simulink model "boost_converter_comparison"  (R2026a)
settings: Solver=ode4  StopTime=0.5  FixedStep=1e-05
values from neighbouring files (symbols this model uses):
  Vref = p.Vref    [disturbance_test_script.m]    (also in run_all_controllers.m)
undefined symbols (not defined in the file or in its folder): C, L, rL, Rload, Vin
libraries: fuzblock x2
settings Model: Creator=akash  LastModifiedBy=akash

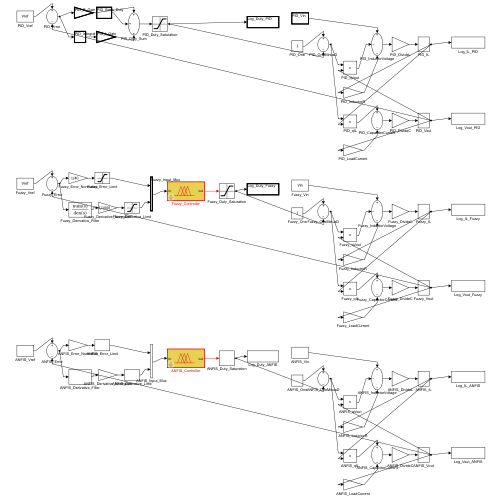
[thumbnail: Simulink's stored preview of the top-level diagram]
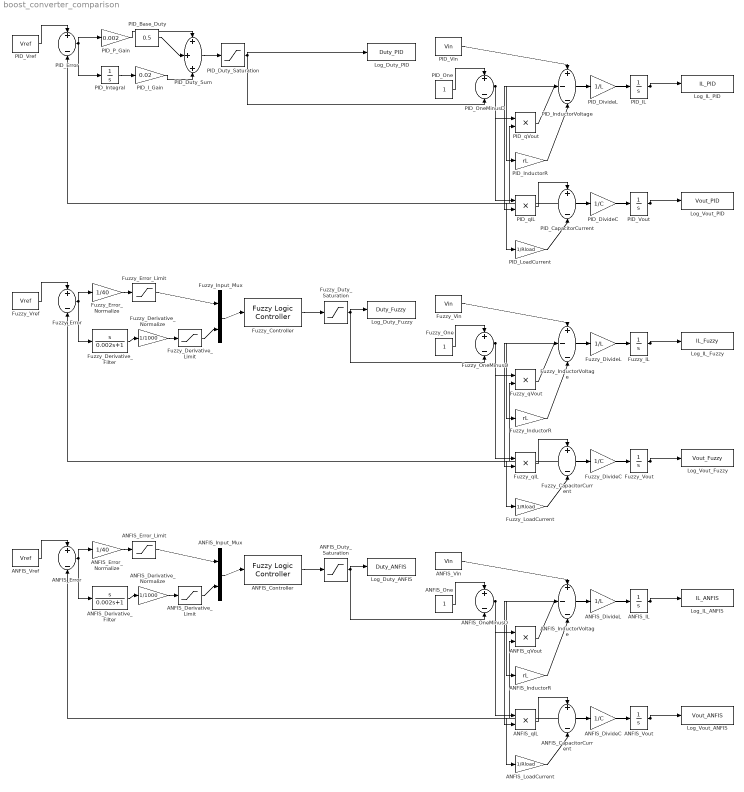
== system boost_converter_comparison ==
  ANFIS_CapacitorCurrent : Sum  Inputs=+-
  ANFIS_Controller : fuzblock/Fuzzy Logic  Controller  FIS=anfisFIS  OutputSampleNumber=101  DataType=double  UseLookupTable=off  NumBreakpoints=10  FuzzifiedInputs=off  RuleFiringStrengths=off  RuleOutputs=off  AggregatedOutputs=off  SimulateUsing=Interpreted execution  OutOfRangeInputValueMessage=warning  NoRuleFiredMessage=warning  EmptyOutputFuzzySetMessage=warning
      settings: LibrarySourceBlock=|
      | fuzblock/Fuzzy Logic
      | Controller
      | with Ruleviewer/Fuzzy Logic
      | Controller
  ANFIS_Derivative_Filter : TransferFcn  Numerator=[1 0]  Denominator=[0.002 1]
  ANFIS_Derivative_Limit : Saturate  UpperLimit=1  LowerLimit=-1
  ANFIS_Derivative_Normalize : Gain  Gain=1/1000
  ANFIS_DivideC : Gain  Gain=1/C
  ANFIS_DivideL : Gain  Gain=1/L
  ANFIS_Duty_Saturation : Saturate  UpperLimit=0.65  LowerLimit=0.35
  ANFIS_Error : Sum  Inputs=+-
  ANFIS_Error_Limit : Saturate  UpperLimit=1  LowerLimit=-1
  ANFIS_Error_Normalize : Gain  Gain=1/40
  ANFIS_IL : Integrator
  ANFIS_InductorR : Gain  Gain=rL
  ANFIS_InductorVoltage : Sum  Inputs=+--
  ANFIS_Input_Mux : Mux  Inputs=2
  ANFIS_LoadCurrent : Gain  Gain=1/Rload
  ANFIS_One : Constant
  ANFIS_OneMinusD : Sum  Inputs=+-
  ANFIS_Vin : Constant  Value=Vin
  ANFIS_Vout : Integrator
  ANFIS_Vref : Constant  Value=Vref
  ANFIS_qIL : Product  Inputs=**
  ANFIS_qVout : Product  Inputs=**
  Fuzzy_CapacitorCurrent : Sum  Inputs=+-
  Fuzzy_Controller : fuzblock/Fuzzy Logic  Controller  FIS=fuzzyFIS  OutputSampleNumber=101  DataType=double  UseLookupTable=off  NumBreakpoints=10  FuzzifiedInputs=off  RuleFiringStrengths=off  RuleOutputs=off  AggregatedOutputs=off  SimulateUsing=Interpreted execution  OutOfRangeInputValueMessage=warning  NoRuleFiredMessage=warning  EmptyOutputFuzzySetMessage=warning
      settings: LibrarySourceBlock=|
      | fuzblock/Fuzzy Logic
      | Controller
      | with Ruleviewer/Fuzzy Logic
      | Controller
  Fuzzy_Derivative_Filter : TransferFcn  Numerator=[1 0]  Denominator=[0.002 1]
  Fuzzy_Derivative_Limit : Saturate  UpperLimit=1  LowerLimit=-1
  Fuzzy_Derivative_Normalize : Gain  Gain=1/1000
  Fuzzy_DivideC : Gain  Gain=1/C
  Fuzzy_DivideL : Gain  Gain=1/L
  Fuzzy_Duty_Saturation : Saturate  UpperLimit=0.65  LowerLimit=0.35
  Fuzzy_Error : Sum  Inputs=+-
  Fuzzy_Error_Limit : Saturate  UpperLimit=1  LowerLimit=-1
  Fuzzy_Error_Normalize : Gain  Gain=1/40
  Fuzzy_IL : Integrator
  Fuzzy_InductorR : Gain  Gain=rL
  Fuzzy_InductorVoltage : Sum  Inputs=+--
  Fuzzy_Input_Mux : Mux  Inputs=2
  Fuzzy_LoadCurrent : Gain  Gain=1/Rload
  Fuzzy_One : Constant
  Fuzzy_OneMinusD : Sum  Inputs=+-
  Fuzzy_Vin : Constant  Value=Vin
  Fuzzy_Vout : Integrator
  Fuzzy_Vref : Constant  Value=Vref
  Fuzzy_qIL : Product  Inputs=**
  Fuzzy_qVout : Product  Inputs=**
  Log_Duty_ANFIS : ToWorkspace  VariableName=Duty_ANFIS  SaveFormat=Timeseries  SampleTime=-1
  Log_Duty_Fuzzy : ToWorkspace  VariableName=Duty_Fuzzy  SaveFormat=Timeseries  SampleTime=-1
  Log_Duty_PID : ToWorkspace  VariableName=Duty_PID  SaveFormat=Timeseries  SampleTime=-1
  Log_IL_ANFIS : ToWorkspace  VariableName=IL_ANFIS  SaveFormat=Timeseries  SampleTime=-1
  Log_IL_Fuzzy : ToWorkspace  VariableName=IL_Fuzzy  SaveFormat=Timeseries  SampleTime=-1
  Log_IL_PID : ToWorkspace  VariableName=IL_PID  SaveFormat=Timeseries  SampleTime=-1
  Log_Vout_ANFIS : ToWorkspace  VariableName=Vout_ANFIS  SaveFormat=Timeseries  SampleTime=-1
  Log_Vout_Fuzzy : ToWorkspace  VariableName=Vout_Fuzzy  SaveFormat=Timeseries  SampleTime=-1
  Log_Vout_PID : ToWorkspace  VariableName=Vout_PID  SaveFormat=Timeseries  SampleTime=-1
  PID_Base_Duty : Constant  Value=0.5
  PID_CapacitorCurrent : Sum  Inputs=+-
  PID_DivideC : Gain  Gain=1/C
  PID_DivideL : Gain  Gain=1/L
  PID_Duty_Saturation : Saturate  UpperLimit=0.65  LowerLimit=0.35
  PID_Duty_Sum : Sum  Inputs=+++
  PID_Error : Sum  Inputs=+-
  PID_IL : Integrator
  PID_I_Gain : Gain  Gain=0.02
  PID_InductorR : Gain  Gain=rL
  PID_InductorVoltage : Sum  Inputs=+--
  PID_Integral : Integrator
  PID_LoadCurrent : Gain  Gain=1/Rload
  PID_One : Constant
  PID_OneMinusD : Sum  Inputs=+-
  PID_P_Gain : Gain  Gain=0.002
  PID_Vin : Constant  Value=Vin
  PID_Vout : Integrator
  PID_Vref : Constant  Value=Vref
  PID_qIL : Product  Inputs=**
  PID_qVout : Product  Inputs=**
  wires:
  PID_Error/1 -> PID_P_Gain/1, PID_Integral/1
  PID_P_Gain/1 -> PID_Duty_Sum/1
  PID_Base_Duty/1 -> PID_Duty_Sum/2
  PID_Integral/1 -> PID_I_Gain/1
  PID_I_Gain/1 -> PID_Duty_Sum/3
  PID_Duty_Sum/1 -> PID_Duty_Saturation/1
  PID_Duty_Saturation/1 -> Log_Duty_PID/1, PID_OneMinusD/2
  PID_Vref/1 -> PID_Error/1
  PID_Vout/1 -> PID_Error/2, PID_qVout/2, PID_LoadCurrent/1, Log_Vout_PID/1
  PID_One/1 -> PID_OneMinusD/1
  PID_OneMinusD/1 -> PID_qVout/1, PID_qIL/1
  PID_IL/1 -> PID_InductorR/1, PID_qIL/2, Log_IL_PID/1
  PID_Vin/1 -> PID_InductorVoltage/1
  PID_qVout/1 -> PID_InductorVoltage/2
  PID_InductorR/1 -> PID_InductorVoltage/3
  PID_InductorVoltage/1 -> PID_DivideL/1
  PID_DivideL/1 -> PID_IL/1
  PID_qIL/1 -> PID_CapacitorCurrent/1
  PID_LoadCurrent/1 -> PID_CapacitorCurrent/2
  PID_CapacitorCurrent/1 -> PID_DivideC/1
  PID_DivideC/1 -> PID_Vout/1
  Fuzzy_Error/1 -> Fuzzy_Error_Normalize/1, Fuzzy_Derivative_Filter/1
  Fuzzy_Error_Normalize/1 -> Fuzzy_Error_Limit/1
  Fuzzy_Derivative_Filter/1 -> Fuzzy_Derivative_Normalize/1
  Fuzzy_Derivative_Normalize/1 -> Fuzzy_Derivative_Limit/1
  Fuzzy_Error_Limit/1 -> Fuzzy_Input_Mux/1
  Fuzzy_Derivative_Limit/1 -> Fuzzy_Input_Mux/2
  Fuzzy_Input_Mux/1 -> Fuzzy_Controller/1
  Fuzzy_Controller/1 -> Fuzzy_Duty_Saturation/1
  Fuzzy_Duty_Saturation/1 -> Log_Duty_Fuzzy/1, Fuzzy_OneMinusD/2
  Fuzzy_Vref/1 -> Fuzzy_Error/1
  Fuzzy_Vout/1 -> Fuzzy_Error/2, Fuzzy_qVout/2, Fuzzy_LoadCurrent/1, Log_Vout_Fuzzy/1
  Fuzzy_One/1 -> Fuzzy_OneMinusD/1
  Fuzzy_OneMinusD/1 -> Fuzzy_qVout/1, Fuzzy_qIL/1
  Fuzzy_IL/1 -> Fuzzy_InductorR/1, Fuzzy_qIL/2, Log_IL_Fuzzy/1
  Fuzzy_Vin/1 -> Fuzzy_InductorVoltage/1
  Fuzzy_qVout/1 -> Fuzzy_InductorVoltage/2
  Fuzzy_InductorR/1 -> Fuzzy_InductorVoltage/3
  Fuzzy_InductorVoltage/1 -> Fuzzy_DivideL/1
  Fuzzy_DivideL/1 -> Fuzzy_IL/1
  Fuzzy_qIL/1 -> Fuzzy_CapacitorCurrent/1
  Fuzzy_LoadCurrent/1 -> Fuzzy_CapacitorCurrent/2
  Fuzzy_CapacitorCurrent/1 -> Fuzzy_DivideC/1
  Fuzzy_DivideC/1 -> Fuzzy_Vout/1
  ANFIS_Error/1 -> ANFIS_Error_Normalize/1, ANFIS_Derivative_Filter/1
  ANFIS_Error_Normalize/1 -> ANFIS_Error_Limit/1
  ANFIS_Derivative_Filter/1 -> ANFIS_Derivative_Normalize/1
  ANFIS_Derivative_Normalize/1 -> ANFIS_Derivative_Limit/1
  ANFIS_Error_Limit/1 -> ANFIS_Input_Mux/1
  ANFIS_Derivative_Limit/1 -> ANFIS_Input_Mux/2
  ANFIS_Input_Mux/1 -> ANFIS_Controller/1
  ANFIS_Controller/1 -> ANFIS_Duty_Saturation/1
  ANFIS_Duty_Saturation/1 -> Log_Duty_ANFIS/1, ANFIS_OneMinusD/2
  ANFIS_Vref/1 -> ANFIS_Error/1
  ANFIS_Vout/1 -> ANFIS_Error/2, ANFIS_qVout/2, ANFIS_LoadCurrent/1, Log_Vout_ANFIS/1
  ANFIS_One/1 -> ANFIS_OneMinusD/1
  ANFIS_OneMinusD/1 -> ANFIS_qVout/1, ANFIS_qIL/1
  ANFIS_IL/1 -> ANFIS_InductorR/1, ANFIS_qIL/2, Log_IL_ANFIS/1
  ANFIS_Vin/1 -> ANFIS_InductorVoltage/1
  ANFIS_qVout/1 -> ANFIS_InductorVoltage/2
  ANFIS_InductorR/1 -> ANFIS_InductorVoltage/3
  ANFIS_InductorVoltage/1 -> ANFIS_DivideL/1
  ANFIS_DivideL/1 -> ANFIS_IL/1
  ANFIS_qIL/1 -> ANFIS_CapacitorCurrent/1
  ANFIS_LoadCurrent/1 -> ANFIS_CapacitorCurrent/2
  ANFIS_CapacitorCurrent/1 -> ANFIS_DivideC/1
  ANFIS_DivideC/1 -> ANFIS_Vout/1
